simulink model "modele_canal_unif"  (R2024b)
settings: Solver=FixedStepDiscrete  StartTime=0.0  StopTime=(Nsim-1)*Tb  FixedStep=Tb  RelTol=1e-3
undefined symbols (not defined in the file or in its folder): a, A, graine, p1, s, Tb
settings Model: Creator=youka  LastModifiedBy=youka

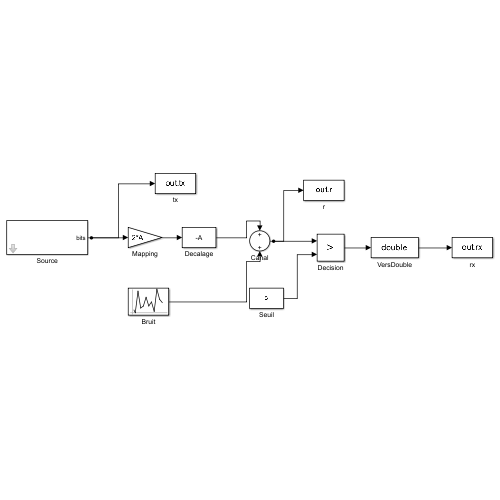
[thumbnail: Simulink's stored preview of the top-level diagram]
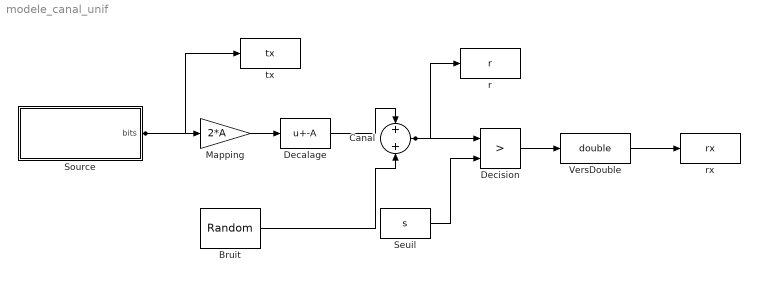
== system modele_canal_unif ==
  Bruit : UniformRandomNumber  Minimum=-a  Maximum=a  Seed=graine+1  SampleTime=Tb
  Canal : Sum
  Decalage : Bias  Bias=-A  SaturateOnIntegerOverflow=off
  Decision : RelationalOperator  Operator=>  OutDataTypeStr=boolean  RndMeth=Simplest  InputSameDT=off
  Mapping : Gain  Gain=2*A
  Seuil : Constant  Value=s  SampleTime=Tb
  Source : Subsystem  mask(Source binaire){p_m=p1, Tb_m=Tb, graine_m=graine}
      mask prompts: p_m "Probabilité d'émettre un 1"; Tb_m "Durée d'un bit Tb (s)"; graine_m "Graine (Seed)"
      mask help: Source binaire sans mémoire : P(1) = p, un bit toutes les Tb secondes.
  VersDouble : DataTypeConversion  OutDataTypeStr=double  SaturateOnIntegerOverflow=off  RndMeth=Floor
  r : ToWorkspace  VariableName=r  SampleTime=-1
  rx : ToWorkspace  VariableName=rx  SampleTime=-1
  tx : ToWorkspace  VariableName=tx  SampleTime=-1
  wires:
  Source/1(bits) -> tx/1, Mapping/1
  Mapping/1 -> Decalage/1
  Decalage/1 -> Canal/1
  Bruit/1 -> Canal/2
  Canal/1 -> Decision/1, r/1
  Seuil/1 -> Decision/2
  Decision/1 -> VersDouble/1
  VersDouble/1 -> rx/1

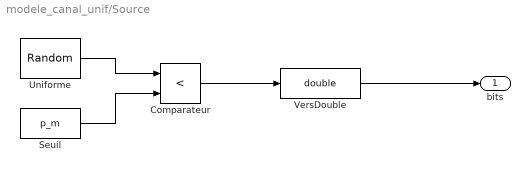
== system modele_canal_unif/Source ==
  Comparateur : RelationalOperator  Operator=<  OutDataTypeStr=boolean  RndMeth=Simplest  InputSameDT=off
  Seuil : Constant  Value=p_m  SampleTime=Tb_m
  Uniforme : UniformRandomNumber  Minimum=0  Seed=graine_m  SampleTime=Tb_m
  VersDouble : DataTypeConversion  OutDataTypeStr=double  SaturateOnIntegerOverflow=off  RndMeth=Floor
  bits : Outport
  wires:
  Uniforme/1 -> Comparateur/1
  Seuil/1 -> Comparateur/2
  Comparateur/1 -> VersDouble/1
  VersDouble/1 -> bits/1
